simulink model "Palan_sim"  (R2019a)
settings: Solver=FixedStepDiscrete  StartTime=0.0  StopTime=inf  FixedStep=2e-4  RelTol=1e-3
PreLoadFcn:
  | waijung.modelPreload; % Required for working with Waijung Blockset. Do not remove.
undefined symbols (not defined in the file): CPHA_1Edge, CPOL_Low, disableTheCustomCode, DISTANCE_PER_TURN_X, Duplex, enableTheCustomCode, FirstBit_MSB, Full, HSEOSC, in1, initTheCustomCode, Link, LQFP64, modifySysTick, out1, outputCSHigh, outputCSLow, PPR_THETA, PPR_XY, PSC2V, ST, STM32F446RE, V2PSC, waitForPulse, xref
libraries: simulink x13, waijung_customcode x4, stm32f4_spi_lib x3, stm32f4_io_lib x2, stm32f4_device_config_lib x1
CloseFcn:
  | waijung.modelClose; % Required for working with Waijung Blockset. Do not remove.
settings Model: Creator=ELEPALAN  LastModifiedBy=ELE4202-200
settings OptimizationCC: DefaultParameterBehavior=Inlined  DefaultUnderspecifiedDataType=single  EnhancedBackFolding=on  PassReuseOutputArgsAs=Individual arguments  ZeroExternalMemoryAtStartup=off  ZeroInternalMemoryAtStartup=off  MaxStackSize=64  OptimizeBlockOrder=speed  DifferentSizesBufferReuse=on  OptimizationCustomize=off
settings DebuggingCC: ParameterTunabilityLossMsg=error  UnconnectedInputMsg=none  UnconnectedOutputMsg=none  UnconnectedLineMsg=none  SFMachineParentedDataDiag=error
settings HardwareCC: ProdBitPerPointer=32  ProdBitPerSizeT=32  ProdBitPerPtrDiffT=32  ProdLargestAtomicInteger=Long  ProdLargestAtomicFloat=Double  ProdWordSize=32  ProdLongLongMode=on  ProdHWDeviceType=ARM Compatible->ARM Cortex  TargetEndianess=LittleEndian
settings SFSimCC: MATLABDynamicMemAlloc=off
settings RTWCC: Description=STM32F4 Target  SystemTargetFile=stm32f4.tlc  GenerateMakefile=off  TemplateMakefile=ert_default_tmf  Toolchain=GNU Tools for ARM Embedded Processors
settings CodeAppCC: ForceParamTrailComments=on  IgnoreCustomStorageClasses=off  OperatorAnnotations=on  SimulinkDataObjDesc=on  SFDataObjDesc=on  InsertBlockDesc=on
settings STFCustomTargetCC: MultiwordLength=256  ModelReferenceCompliant=off  CombineOutputUpdateFcns=on  ERTCustomFileBanners=on  SupportContinuousTime=off  SupportNonInlinedSFcns=off  RemoveResetFunc=on  MATLABClassNameForMDSCustomization=Simulink.SoftwareTarget.ERTCustomization  GRTInterface=off  SystemTargetFile=stm32f4.tlc
settings ERTTargetCC: ModelReferenceCompliant=off  ParMdlRefBuildCompliant=off  CompOptLevelCompliant=off  ConcurrentExecutionCompliant=off  ModelStepFunctionPrototypeControlCompliant=off  CPPClassGenCompliant=off  UseToolchainInfoCompliant=off  InlinedParameterPlacement=NonHierarchical  ERTSrcFileBannerTemplate=stm32f4_code_template.cgt  ERTHdrFileBannerTemplate=stm32f4_code_template.cgt  ERTDataSrcFileTemplate=stm32f4_code_template.cgt  ERTDataHdrFileTemplate=stm32f4_code_template.cgt  ERTCustomFileTemplate=stm32f4_file_process.tlc

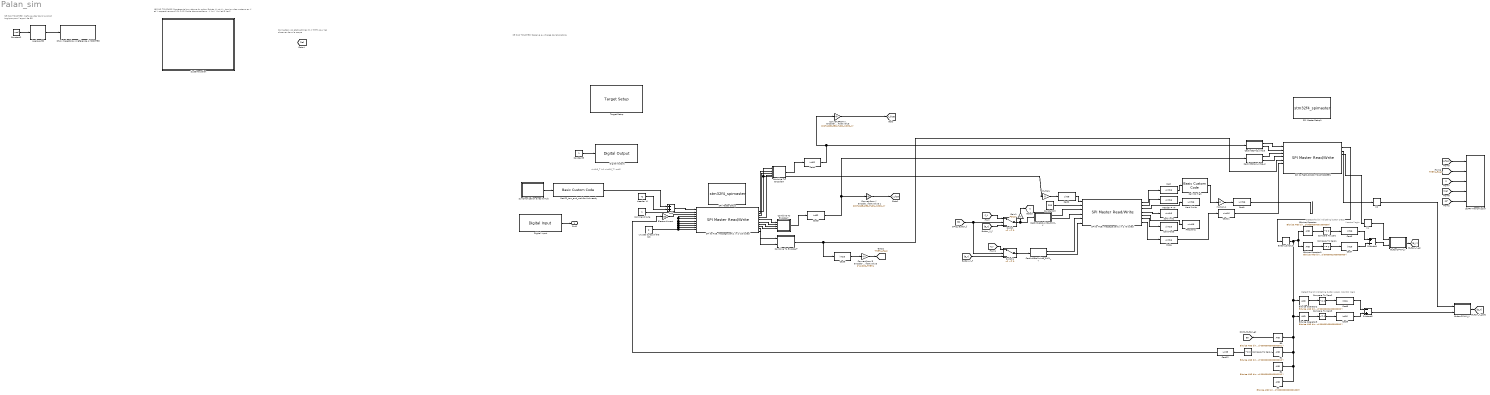
== system Palan_sim ==
  note: Detect the bit indicating button press.
  note: uint16_T in1,uint16_T* out1)
  note: NE PAS TOUCHER! Réservé au chargé de laboratoire
  note: Detect the bit indicating button press.
  note: Ycontrol logic
  note: Xcontrol logic
  note: NE PAS TOUCHER!
      | Xref à ajuster dans le script
      | Logique pour l'appui de B0
  note: Connectez vos états estimés [X,X',θ,θ'] pour les
      | observer dans le scope
  note: NE PAS TOUCHER!
      | Représente le système du palan
      | Entrée Vx et Vy: tension des moteurs en X et Y respectivement [-24,24]V
      | Sortie des encodeurs : X (m), Y(m) et θ (rad)
  Add : Sum  OutDataTypeStr=uint8  SaturateOnIntegerOverflow=on  InputSameDT=on
  B0 : simulink/Logic and Bit Operations/Bitwise Operator  logicop=AND  UseBitMask=on  BitMask=bin2dec('0000000000000001')  BitMaskRealWorld=Stored Integer
  B1 : simulink/Logic and Bit Operations/Bitwise Operator  logicop=AND  UseBitMask=on  BitMask=bin2dec('0000000000000010')  BitMaskRealWorld=Stored Integer
  B2 : simulink/Logic and Bit Operations/Bitwise Operator  logicop=AND  UseBitMask=on  BitMask=bin2dec('0000000000000100')  BitMaskRealWorld=Stored Integer
  B3 : simulink/Logic and Bit Operations/Bitwise Operator  logicop=AND  UseBitMask=on  BitMask=bin2dec('0000000000001000')  BitMaskRealWorld=Stored Integer
  Bitwise Operator : simulink/Logic and Bit Operations/Bitwise Operator  logicop=AND  UseBitMask=on  BitMask=bin2dec('0000000001000000')  BitMaskRealWorld=Stored Integer
  Bitwise Operator1 : simulink/Logic and Bit Operations/Bitwise Operator  logicop=AND  UseBitMask=on  BitMask=bin2dec('0000001000000000')  BitMaskRealWorld=Stored Integer
  Bitwise Operator2 : simulink/Logic and Bit Operations/Bitwise Operator  logicop=AND  UseBitMask=on  BitMask=bin2dec('0000000100000000')  BitMaskRealWorld=Stored Integer
  Bitwise Operator3 : simulink/Logic and Bit Operations/Bitwise Operator  logicop=AND  UseBitMask=on  BitMask=bin2dec('0000010000000000')  BitMaskRealWorld=Stored Integer
  Button2PWM_X : MATLAB Function  TreatAsAtomicUnit=on
  Button2PWM_Y : MATLAB Function  TreatAsAtomicUnit=on
  Button_Outputs : Memory
  CalibMode : DataTypeConversion  OutDataTypeStr=uint16
  Call CS High : waijung_customcode/Basic Custom Code  inputporttype=uint16  cinputportlabel=in1  cinputportlabelstr="[\"in1\"]"  inputportcount=1  inputporttypeid=[5]  outputporttype=uint16  coutputportlabel=ForceMeFirst  coutputportlabelstr="[\"ForceMeFirst\"]"  outputportcount=1  outputporttypeid=[5]  incpath={}  srcpath={fullfile(pwd,'customcode')}  incfiles={}  srcfiles={'customcode.c'}  initialfuncallstr=initTheCustomCode();  enablefuncallstr=enableTheCustomCode();  outputfuncallstr=outputCSHigh(in1,out1);  disablefuncallstr=disableTheCustomCode();  sampletime=2e-4  sampletimestr=-1  blockid=CallCSHigh  enablecustomportlabel=on  incfilestrarray=[]  inputportdiminfo="[1  1  1  5]"  outputportdiminfo="[1  1  1  5]"
      settings: SourceProductName=Waijung Blockset
  Cast : DataTypeConversion  OutDataTypeStr=uint16
  Cast1 : DataTypeConversion  OutDataTypeStr=uint16
  Cast11 : DataTypeConversion  OutDataTypeStr=uint16
  Cast12 : DataTypeConversion  OutDataTypeStr=uint8
  Cast2 : DataTypeConversion  OutDataTypeStr=uint8
  Cast{3,6..9} (5 alike) : DataTypeConversion  OutDataTypeStr=int16
  Cast4 : DataTypeConversion  OutDataTypeStr=int32
  Cast5 : DataTypeConversion  OutDataTypeStr=int32
  Castint16to2uint8_PWM_X : MATLAB Function  TreatAsAtomicUnit=on
  Castint16to2uint8_PWM_Y : MATLAB Function  TreatAsAtomicUnit=on
  Castint32To2uint16 : MATLAB Function  TreatAsAtomicUnit=on
  Castint32to2uint16_2 : MATLAB Function  TreatAsAtomicUnit=on
  Choix trajectoire vs référence À MODIFIER : Subsystem
  Combine To EncoderT : MATLAB Function  TreatAsAtomicUnit=on
  Combine To EncoderX : MATLAB Function  TreatAsAtomicUnit=on
  Combine To EncoderY : MATLAB Function  TreatAsAtomicUnit=on
  Commend byte : Constant  OutDataTypeStr=uint8  SampleTime=2e-4
  Compare To Zero{,1..4} (5 alike) : simulink/Logic and Bit Operations/Compare To Zero  relop=~=  OutDataTypeStr=boolean
  Constant13 : Constant  Value=255  OutDataTypeStr=uint8  SampleTime=2e-4
  Constant2 : Constant  Value=xref  SampleTime=-1
  Constant5 : Constant  OutDataTypeStr=boolean  SampleTime=2e-4
  "Convert FROM X encoder to X float value " : Gain  Gain=DISTANCE_PER_TURN_X/PPR_XY  OutDataTypeStr=single  SaturateOnIntegerOverflow=on  ParamDataTypeStr=Inherit: Same as input
  Convert from Y encoder to Y float value 1 : Gain  Gain=DISTANCE_PER_TURN_X/PPR_XY  OutDataTypeStr=single  SaturateOnIntegerOverflow=on  ParamDataTypeStr=Inherit: Same as input
  Convert from θ encoder to θ float value : Gain  Gain=2*pi/PPR_THETA  OutDataTypeStr=single  SaturateOnIntegerOverflow=on  ParamDataTypeStr=Inherit: Same as input
  Digital Input : stm32f4_io_lib/Digital Input  port=A  speed=100  porttype=None  porttypestr=NOPULL  use_pin0=on  use_pin1=off  use_pin2=off  use_pin3=off  use_pin4=off  use_pin5=off  use_pin6=off  use_pin7=off  use_pin8=off  use_pin9=off  use_pin10=off  use_pin11=off  use_pin12=off  use_pin13=off  use_pin14=off  use_pin15=off  pinstr=GPIO_Pin_0  usedpinarray="[1  0  0  0  0  0  0  0  0  0  0  0  0  0  0  0]"  bitbandingstr="#define DigitalInput_A0 Peripheral_BB(GPIOA->IDR, 0)  /* Output pin */"  sampletime=2e-4  sampletimestr=-1  blockid=DigitalInput  enablecustomportlabel=off  glabalinit=off  cinputportlabel=In1, In2  coutputportlabel=Out1, Out2
      settings: SourceProductName=Waijung Blockset
  Digital Output : stm32f4_io_lib/Digital Output  use_bitband=on  port=A  speed=100  porttype=Push Pull  porttypestr=PP  use_pin0=off  use_pin1=off  use_pin2=off  use_pin3=off  use_pin4=off  use_pin5=off  use_pin6=off  use_pin7=off  use_pin8=off  use_pin9=off  use_pin10=on  use_pin11=off  use_pin12=off  use_pin13=off  use_pin14=off  use_pin15=off  pinstr=GPIO_Pin_10  usedpinarray="[0  0  0  0  0  0  0  0  0  0  1  0  0  0  0  0]"  bitbandingstr="#define DigitalOutput_A10 Peripheral_BB(GPIOA->ODR, 10)  /* Output pin */"  sampletime=-1  sampletimestr=-1  blockid=DigitalOutput  enablecustomportlabel=off  globalinit=off  cinputportlabel=In1, In2  coutputportlabel=0
      settings: SourceProductName=Waijung Blockset
  Electro-Aimant : Gain  Gain=100  OutDataTypeStr=uint8  SaturateOnIntegerOverflow=on  ParamDataTypeStr=Inherit: Same as input
  Frequency : DataTypeConversion  OutDataTypeStr=uint16
  Gain1 : Gain  Gain=PSC2V  SaturateOnIntegerOverflow=on  OutDataTypeStr=Inherit: Same as input  ParamDataTypeStr=Inherit: Same as input
  Hard limits : DataTypeConversion  OutDataTypeStr=uint16
  Header 'H' : Constant  Value=72  OutDataTypeStr=uint8  SampleTime=2e-4
  Header = 'H' : DataTypeConversion  OutDataTypeStr=uint16
  K0 : Memory
  K1 : Memory
  Logique B0 : Subsystem
  Mode : DataTypeConversion  OutDataTypeStr=uint16
  Multiply : Gain  Gain=0  SaturateOnIntegerOverflow=on  OutDataTypeStr=Inherit: Same as input  ParamDataTypeStr=Inherit: Same as input
  Multiply1 : Gain  Gain=0  SaturateOnIntegerOverflow=on  OutDataTypeStr=Inherit: Same as input  ParamDataTypeStr=Inherit: Same as input
  SPI Master Setup : S-Function  FunctionName=stm32f4_spimaster  Parameters=mode,configuration,module,datacount,inputtypearray,outputtypearray,confstr,sampletime,sampletimestr,blockid  SFunctionDeploymentMode=off  EnableBusSupport=off  mask(stm32f4_spimaster){configuration=Setup, module=3, mode=Write, lastmodule=3, direction=Full-Duplex, dataformat=8bit/ FirstBit_MSB, prescaler=8, lastpclk=45000000, baudrate=5625000, cpolcpha=CPOL_Low/ CPHA_1Edge, datacount=0, nssmode=Software, nsspin=Not used, softnssport=B, softnsspin=10, sckpin=B3, misopin=B4, mosipin=B5, pintype=Push Pull, pulltype=None, nssdelay=0, inputtypearray=[0], outputtypearray=[0], confstr=["SPI_Direction_2Lines_FullDuplex","8b","MSB","Low","1Edge","8","Soft","0","x","x","1","B","10","1","B","3","1","B","4","1","B","5","0","1","0","0","0","0","0","0","0","PP","0","NOPULL"], sampletime=-1, sampletimestr=-1, blockid=SPIMasterSetup}
      mask prompts: module "SPI Module:"; lastmodule "Last module:"; dataformat "Data format:"; prescaler "Buad rate prescaler: Pclk/"; lastpclk "Last PCLK"; baudrate "Baud rate (Hz)"; cpolcpha "Clock polarity (CPOL)/ Clock phase (CPHA):"; datacount "Data Write count:"; nssmode "Slave/chip select (nSS, nCS) mode"; nsspin "Slave/chip select (nSS, nCS) pin"; softnssport "Slave/chip select port (nSS, nCS)"; softnsspin "Slave/chip select pin (nSS, nCS)"; sckpin "SCLK pin:"; misopin "MISO pin:"; mosipin "MOSI pin:"; pintype "Pin type (Push-Pull/Open-Drain)"; pulltype "Pull Type (Up/Down)"; nssdelay "Data delay time, uS:"; inputtypearray "Input type array"; outputtypearray "Output type array"; confstr "Configuration string"; sampletime "Sample time (sec)"; sampletimestr "Compiled sample time (sec) in string"
      mask help:
      | Direction:
      |  - Full-Duplex, use this mode when need to send and receive data at same clock.
      |  - Half-Duplex_Tx, this mode is to transmit data to slave only. Pin MISO (Rx) can be free for other function.
      |  - Half-Duplex_Rx, this mode is to receive data from slave only. Pin MOSIO (Tx) can be free for other function.
      | Data format:
      |   This configuration is depending on the specification of slave device.
      | Baud rate prescaler:
      |  - Use this prescaler to devide from the PCLK for SPI clock.
      |  - This Prescaler value is auto determine corresponding to baudrate setting and selected SPI module.
      | Baud rate (Hz):
      |  - Select baud rate for SPI clock. Please check the maximum clock support for target slave device.
      | Clock polarity and Clock phase:
      |  - This configuration parameter is depending on slave device.
      |  - See waijung help for more description.
      | Slave/chip select mode:
      |  - Hardware, use hardware SPI module for slave select (or chip select) pin.
      |  - Software, this mode allow any available pin for slave select (or chip select) function.
      |  - Custom, SPI block did not control slave select pin. User may use Digital Output block to control by costom.
      mask init:
      | stm32f4_spimaster_callback('init');
      mask Help: web(fullfile(waijungdocroot,'stm32f4_spimaster_setup.htm'), '-browser')
      mask TypeOptions configuration: Setup | Transaction
      mask Callback configuration: stm32f4_spimaster_callback('configuration');
      mask TypeOptions module: 1 | 2 | 3
      mask Callback module: stm32f4_spimaster_callback('module');
      mask TypeOptions mode: Read/ Write | Read | Write
      mask Callback mode: stm32f4_spimaster_callback('mode');
      mask TypeOptions direction: Full-Duplex | Half-Duplex_Tx | Half-Duplex_Rx
      mask Callback direction: stm32f4_spimaster_callback('direction');
      mask TypeOptions dataformat: 8bit/ FirstBit_MSB | 8bit/ FirstBit_LSB | 16bit/ FirstBit_MSB | 16bit/ FirstBit_LSB
      mask TypeOptions prescaler: 2 | 4 | 8 | 16 | 32 | 64 | 128 | 256
      mask TypeOptions baudrate: Not set | 22500000 | 11250000 | 5625000 | 2812500 | 1406250 | 703125 | 351563 | 175781
      mask Callback baudrate: stm32f4_spimaster_callback('baudrate');
      mask TypeOptions cpolcpha: CPOL_Low/ CPHA_1Edge | CPOL_Low/ CPHA_2Edge | CPOL_High/ CPHA_1Edge | CPOL_High/ CPHA_2Edge
      mask Callback datacount: stm32f4_spimaster_callback('datacount');
      mask TypeOptions nssmode: Hardware | Software | Custom
      mask Callback nssmode: stm32f4_spimaster_callback('nssmode');
      mask TypeOptions nsspin: Not used | A4
      mask TypeOptions softnssport: A | B | C | D | E | F | G | H | I
      mask TypeOptions softnsspin: 0 | 1 | 2 | 3 | 4 | 5 | 6 | 7 | 8 | 9 | 10 | 11 | 12 | 13 | 14 | 15
      mask TypeOptions sckpin: Not used | B3 | C10
      mask TypeOptions misopin: Not used | B4 | C11
      mask TypeOptions mosipin: Not used | B5 | C12
      mask TypeOptions pintype: Push Pull | Open Drain
      mask TypeOptions pulltype: None | Pull Up | Pull Down
      mask Callback confstr: stm32f4_spimaster_callback('confstr');
      mask Callback sampletime: stm32f4_spimaster_callback('sampletime');
      mask Callback sampletimestr: stm32f4_spimaster_callback('sampletimestr');
      mask Callback blockid: stm32f4_spimaster_callback('blockid');
      mask Display: text(0.5, 0.5, 'Module: SPI3 (Master)\nFull-Duplex\nBaudrate: 5625000','ver','middle','hor','center');
  SPI Master Setup1 : S-Function  FunctionName=stm32f4_spimaster  Parameters=mode,configuration,module,datacount,inputtypearray,outputtypearray,confstr,sampletime,sampletimestr,blockid  SFunctionDeploymentMode=off  EnableBusSupport=off  mask(stm32f4_spimaster){configuration=Setup, module=1, mode=Write, lastmodule=1, direction=Full-Duplex, dataformat=16bit/ FirstBit_MSB, prescaler=8, lastpclk=90000000, baudrate=11250000, cpolcpha=CPOL_Low/ CPHA_1Edge, datacount=0, nssmode=Software, nsspin=Not used, softnssport=B, softnsspin=6, sckpin=A5, misopin=A6, mosipin=A7, pintype=Push Pull, pulltype=Pull Up, nssdelay=0, inputtypearray=[0], outputtypearray=[0], confstr=["SPI_Direction_2Lines_FullDuplex","16b","MSB","Low","1Edge","8","Soft","0","x","x","1","B","6","1","A","5","1","A","6","1","A","7","1","1","0","0","0","0","0","0","0","PP","0","UP"], sampletime=-1, sampletimestr=-1, blockid=SPIMasterSetup1}
      mask prompts: module "SPI Module:"; lastmodule "Last module:"; dataformat "Data format:"; prescaler "Buad rate prescaler: Pclk/"; lastpclk "Last PCLK"; baudrate "Baud rate (Hz)"; cpolcpha "Clock polarity (CPOL)/ Clock phase (CPHA):"; datacount "Data Write count:"; nssmode "Slave/chip select (nSS, nCS) mode"; nsspin "Slave/chip select (nSS, nCS) pin"; softnssport "Slave/chip select port (nSS, nCS)"; softnsspin "Slave/chip select pin (nSS, nCS)"; sckpin "SCLK pin:"; misopin "MISO pin:"; mosipin "MOSI pin:"; pintype "Pin type (Push-Pull/Open-Drain)"; pulltype "Pull Type (Up/Down)"; nssdelay "Data delay time, uS:"; inputtypearray "Input type array"; outputtypearray "Output type array"; confstr "Configuration string"; sampletime "Sample time (sec)"; sampletimestr "Compiled sample time (sec) in string"
      mask help:
      | Direction:
      |  - Full-Duplex, use this mode when need to send and receive data at same clock.
      |  - Half-Duplex_Tx, this mode is to transmit data to slave only. Pin MISO (Rx) can be free for other function.
      |  - Half-Duplex_Rx, this mode is to receive data from slave only. Pin MOSIO (Tx) can be free for other function.
      | Data format:
      |   This configuration is depending on the specification of slave device.
      | Baud rate prescaler:
      |  - Use this prescaler to devide from the PCLK for SPI clock.
      |  - This Prescaler value is auto determine corresponding to baudrate setting and selected SPI module.
      | Baud rate (Hz):
      |  - Select baud rate for SPI clock. Please check the maximum clock support for target slave device.
      | Clock polarity and Clock phase:
      |  - This configuration parameter is depending on slave device.
      |  - See waijung help for more description.
      | Slave/chip select mode:
      |  - Hardware, use hardware SPI module for slave select (or chip select) pin.
      |  - Software, this mode allow any available pin for slave select (or chip select) function.
      |  - Custom, SPI block did not control slave select pin. User may use Digital Output block to control by costom.
      mask init:
      | stm32f4_spimaster_callback('init');
      mask Help: web(fullfile(waijungdocroot,'stm32f4_spimaster_setup.htm'), '-browser')
      mask TypeOptions configuration: Setup | Transaction
      mask Callback configuration: stm32f4_spimaster_callback('configuration');
      mask TypeOptions module: 1 | 2 | 3
      mask Callback module: stm32f4_spimaster_callback('module');
      mask TypeOptions mode: Read/ Write | Read | Write
      mask Callback mode: stm32f4_spimaster_callback('mode');
      mask TypeOptions direction: Full-Duplex | Half-Duplex_Tx | Half-Duplex_Rx
      mask Callback direction: stm32f4_spimaster_callback('direction');
      mask TypeOptions dataformat: 8bit/ FirstBit_MSB | 8bit/ FirstBit_LSB | 16bit/ FirstBit_MSB | 16bit/ FirstBit_LSB
      mask TypeOptions prescaler: 2 | 4 | 8 | 16 | 32 | 64 | 128 | 256
      mask TypeOptions baudrate: Not set | 45000000 | 22500000 | 11250000 | 5625000 | 2812500 | 1406250 | 703125 | 351563 | 5250000
      mask Callback baudrate: stm32f4_spimaster_callback('baudrate');
      mask TypeOptions cpolcpha: CPOL_Low/ CPHA_1Edge | CPOL_Low/ CPHA_2Edge | CPOL_High/ CPHA_1Edge | CPOL_High/ CPHA_2Edge
      mask Callback datacount: stm32f4_spimaster_callback('datacount');
      mask TypeOptions nssmode: Hardware | Software | Custom
      mask Callback nssmode: stm32f4_spimaster_callback('nssmode');
      mask TypeOptions nsspin: Not used | A4 | A15
      mask TypeOptions softnssport: A | B | C | D | E | F | G | H | I
      mask TypeOptions softnsspin: 0 | 1 | 2 | 3 | 4 | 5 | 6 | 7 | 8 | 9 | 10 | 11 | 12 | 13 | 14 | 15
      mask TypeOptions sckpin: Not used | A5 | B3
      mask TypeOptions misopin: Not used | A6 | B4
      mask TypeOptions mosipin: Not used | A7 | B5
      mask TypeOptions pintype: Push Pull | Open Drain
      mask TypeOptions pulltype: None | Pull Up | Pull Down
      mask Callback confstr: stm32f4_spimaster_callback('confstr');
      mask Callback sampletime: stm32f4_spimaster_callback('sampletime');
      mask Callback sampletimestr: stm32f4_spimaster_callback('sampletimestr');
      mask Callback blockid: stm32f4_spimaster_callback('blockid');
      mask Display: text(0.5, 0.5, 'Module: SPI1 (Master)\nFull-Duplex\nBaudrate: 11250000','ver','middle','hor','center');
  SPI to F469I-DISCO TOUCHSCREEN : stm32f4_spi_lib/SPI Master Read//Write  configuration=Transaction  module=1  mode=Read/ Write  lastmodule=1  direction=Full-Duplex  dataformat=16bit/ FirstBit_MSB  prescaler=4  cpolcpha=CPOL_Low/ CPHA_1Edge  datacount=8  nssmode=Custom  nsspin=Not used  softnssport=E  softnsspin=0  sckpin=A5  misopin=A6  mosipin=A7  inputtypearray=[8 5 5 5 5 5 5 5 5]  outputtypearray=[9 7 5 5 5 5 5 5 5 5]  confstr="[\"SPI_Direction_2Lines_FullDuplex\",\"16b\",\"MSB\",\"Low\",\"1Edge\",\"4\",\"Soft\",\"0\",\"x\",\"x\",\"0\",\"x\",\"x\",\"1\",\"A\",\"5\",\"1\",\"A\",\"6\",\"1\",\"A\",\"7\",\"1\",\"0\",\"0\",\"0\",\"0\",\"0\",\"0\",\"0\",\"0\",\"PP\",\"0\",\"UP\"]"  sampletime=2e-4  sampletimestr=-1  blockid=SPItoF469IDISCOTOUCHSCREEN
      settings: SourceProductName=Waijung Blockset
  "SPI to HUB, message part 1 in 2 (10 bytes)" : stm32f4_spi_lib/SPI Master Read//Write  configuration=Transaction  module=3  mode=Read/ Write  lastmodule=1  direction=Full-Duplex  dataformat=8bit/ FirstBit_MSB  prescaler=4  cpolcpha=CPOL_Low/ CPHA_1Edge  datacount=10  nssmode=Custom  nsspin=Not used  softnssport=E  softnsspin=0  sckpin=A5  misopin=A6  mosipin=A7  inputtypearray=[10 3 3 3 3 3 3 3 3 3 3]  outputtypearray=[11 7 3 3 3 3 3 3 3 3 3 3]  confstr="[\"SPI_Direction_2Lines_FullDuplex\",\"8b\",\"MSB\",\"Low\",\"1Edge\",\"4\",\"Soft\",\"0\",\"x\",\"x\",\"0\",\"x\",\"x\",\"1\",\"A\",\"5\",\"1\",\"A\",\"6\",\"1\",\"A\",\"7\",\"1\",\"0\",\"0\",\"0\",\"0\",\"0\",\"0\",\"0\",\"0\",\"PP\",\"0\",\"UP\"]"  sampletime=2e-4  sampletimestr=-1  blockid=SPItoHUBmessagepart1in210bytes
      settings: SourceProductName=Waijung Blockset
  "SPI to HUB, message part 2 in 2 (6 bytes)" : stm32f4_spi_lib/SPI Master Read//Write  configuration=Transaction  module=3  mode=Read/ Write  lastmodule=1  direction=Full-Duplex  dataformat=8bit/ FirstBit_MSB  prescaler=4  cpolcpha=CPOL_Low/ CPHA_1Edge  datacount=6  nssmode=Custom  nsspin=Not used  softnssport=E  softnsspin=0  sckpin=A5  misopin=A6  mosipin=A7  inputtypearray=[6 3 3 3 3 3 3]  outputtypearray=[7 7 3 3 3 3 3 3]  confstr="[\"SPI_Direction_2Lines_FullDuplex\",\"8b\",\"MSB\",\"Low\",\"1Edge\",\"4\",\"Soft\",\"0\",\"x\",\"x\",\"0\",\"x\",\"x\",\"1\",\"A\",\"5\",\"1\",\"A\",\"6\",\"1\",\"A\",\"7\",\"1\",\"0\",\"0\",\"0\",\"0\",\"0\",\"0\",\"0\",\"0\",\"PP\",\"0\",\"UP\"]"  sampletime=2e-4  sampletimestr=-1  blockid=SPItoHUBmessagepart2in26bytes
      settings: SourceProductName=Waijung Blockset
  Set CS_Low_and_wait for Hub ready : waijung_customcode/Basic Custom Code  inputporttype=uint16  cinputportlabel=in1  cinputportlabelstr="[\"in1\"]"  inputportcount=1  inputporttypeid=[5]  outputporttype=uint16  coutputportlabel=ForceMeFirst  coutputportlabelstr="[\"ForceMeFirst\"]"  outputportcount=1  outputporttypeid=[5]  incpath={}  srcpath={fullfile(pwd,'customcode')}  incfiles={}  srcfiles={'customcode.c'}  initialfuncallstr=initTheCustomCode();  enablefuncallstr=enableTheCustomCode();  outputfuncallstr=outputCSLow(in1, out1);  disablefuncallstr=disableTheCustomCode();  sampletime=2e-4  sampletimestr=-1  blockid=SetCS_Low_and_waitforHubready  enablecustomportlabel=on  incfilestrarray=[]  inputportdiminfo="[1  1  1  5]"  outputportdiminfo="[1  1  1  5]"
      settings: SourceProductName=Waijung Blockset
  Soft limits : DataTypeConversion  OutDataTypeStr=uint16
  Subtract1 : Sum  Inputs=+-  SaturateOnIntegerOverflow=on  InputSameDT=on  OutDataTypeStr=Inherit: Same as first input
  Subtract2 : Sum  Inputs=-+  SaturateOnIntegerOverflow=on  InputSameDT=on  OutDataTypeStr=Inherit: Same as first input
  Switch : Switch  Criteria=u2 ~= 0  OutDataTypeStr=int32
  Switch1 : Switch  Criteria=u2 ~= 0  OutDataTypeStr=int32
  Synchronisation avec le Hub : Subsystem
  Système palan : Subsystem
  Target Setup : stm32f4_device_config_lib/Target Setup  Priority=100  compiler=GNU ARM  previous_compiler=GNU ARM  mcu=STM32F446RE (LQFP64)  mcustr=STM32F446RE  clockconfig=HSEOSC-8MHz  system_stm32f4xx_c_path=C:\Palans\workspace\ELE3200_Banc_Moteur\waijung_18.11a\targets\stm32f4_target\stm32f4\utils\system_stm32f4xx_default\STM32F446xx\hseosc8mhz  showmemoryconfiguration=off  stacksize=0x2000  heapsize=0x2000  enableautocompiledownload=on  fullchiperase=off  programmerinterface=ST-Link  editctrlstr=on  compilercontrolstr=$(patsubst %, -I%, .) -mcpu=cortex-m4 -mthumb -mthumb-interwork -mfloat-abi=hard -mfpu=fpv4-sp-d16 -ffast-math -Wall -Wextra -Ofast  assemblercontrolstr=$(patsubst %, -I%, .) -mcpu=cortex-m4 -mthumb -mthumb-interwork -mfloat-abi=hard -mfpu=fpv4-sp-d16 -ffast-math -Wall -Wextra -Ofast -Wa,-amhls=$(<:.s=.lst) -D__STACK_SIZE=$(STACK_SIZE) -D__HEAP_SIZE=$(HEAP_SIZE)  linkercontrolstr=-T$(LD_SCRIPT) -g -Wl,-Map=$(MAP),--cref,--no-warn-mismatch -mcpu=cortex-m4 -mthumb -mthumb-interwork -mfloat-abi=hard -mfpu=fpv4-sp-d16 -specs=nosys.specs  runafterdownload=on  execprofile=None  profileruart=2  profilerbaud=500000  profilertxpin=A2  profilerinitstr=2e-4,180000000,36000,500000,0  manualsetsampletime=on  sampletime=2e-4  blockid=TargetSetup  systickreloadvalue=36000  hseval=8000000  lastprofileruart=2  hclk=180000000  flashorigin=0x8000000  flashlength=512k  ramorigin=0x20000000  ramlength=128k  useextram=off
      settings: SourceProductName=Waijung Blockset
  USART Transmission : Subsystem  Description="Blok envoyant les données par UART pour qu'elles soient lues et enregistrées par l'ordianteur via le modèle simulink \"Host\""
  unused bytes of the SPI : Constant  Value=0  OutDataTypeStr=uint8  SampleTime=2e-4
  Out1 : Outport
  tag scope: B0=global, THETA_float=global, U=global, X_float=global, Y_float=global
  wires:
  Digital Input/1 -> Out1/1
  Subtract1/1 -> Button2PWM_Y/2(u)
  SPI to F469I-DISCO TOUCHSCREEN/3 -> K0/1
  "SPI to HUB, message part 1 in 2 (10 bytes)"/2 -> Combine To EncoderX/1(u1), Multiply/1
  [B_X] -> Switch/3
  Combine To EncoderX/1(x) -> Cast4/1
  "SPI to HUB, message part 2 in 2 (6 bytes)"/1 -> Cast/1
  Convert from θ encoder to θ float value/1 -> [THETA_float]
  Compare To Zero3/1 -> Cast9/1
  Button2PWM_Y/1(y) -> [B_Y]
  B0/1 -> [B0]
  "SPI to HUB, message part 1 in 2 (10 bytes)"/4 -> Combine To EncoderX/3(u3)
  Castint16to2uint8_PWM_X/2(x2) -> "SPI to HUB, message part 2 in 2 (6 bytes)"/4
  Castint32to2uint16_2/2(y) -> SPI to F469I-DISCO TOUCHSCREEN/4
  Cast1/1 -> ?
  "SPI to HUB, message part 1 in 2 (10 bytes)"/3 -> Combine To EncoderX/2(u2)
  [F_Y] -> Switch1/1
  "Convert FROM X encoder to X float value "/1 -> [X_float]
  [B_Y] -> Switch1/3
  Cast7/1 -> Subtract1/2
  Multiply1/1 -> Cast1/1
  B1/1 -> Compare To Zero4/1
  Castint16to2uint8_PWM_Y/1(x1) -> "SPI to HUB, message part 2 in 2 (6 bytes)"/5
  Cast12/1 -> Electro-Aimant/1
  Bitwise Operator3/1 -> Compare To Zero3/1
  Header 'H'/1 -> Add/2
  Compare To Zero/1 -> Cast3/1
  Combine To EncoderT/1(x) -> SPI to F469I-DISCO TOUCHSCREEN/5, Cast6/1
  Multiply/1 -> Cast2/1
  Constant5/1 -> Digital Output/1
  "SPI to HUB, message part 1 in 2 (10 bytes)"/8 -> Combine To EncoderY/3(u3)
  Combine To EncoderY/1(x) -> Cast5/1
  "SPI to HUB, message part 1 in 2 (10 bytes)"/9 -> Combine To EncoderY/4(u4)
  "SPI to HUB, message part 2 in 2 (6 bytes)"/3 -> Hard limits/1
  "SPI to HUB, message part 1 in 2 (10 bytes)"/11 -> Combine To EncoderT/2(u2)
  Cast3/1 -> Subtract1/1
  "SPI to HUB, message part 2 in 2 (6 bytes)"/6 -> CalibMode/1
  Set CS_Low_and_wait for Hub ready/1 -> Add/1  "0"
  "SPI to HUB, message part 2 in 2 (6 bytes)"/5 -> Frequency/1
  SPI to F469I-DISCO TOUCHSCREEN/2 -> Button_Outputs/1
  Button_Outputs/1 -> Bitwise Operator/1, Bitwise Operator1/1, B2/1, B3/1, B1/1, B0/1, Bitwise Operator3/1, Bitwise Operator2/1
  "SPI to HUB, message part 2 in 2 (6 bytes)"/2 -> Header = 'H'/1
  Cast2/1 -> "SPI to HUB, message part 2 in 2 (6 bytes)"/1
  K0/1 -> Button2PWM_X/1(K)
  "SPI to HUB, message part 1 in 2 (10 bytes)"/5 -> Combine To EncoderX/4(u4)
  Button2PWM_X/1(y) -> [B_X]
  Bitwise Operator1/1 -> Compare To Zero1/1
  Cast5/1 -> Castint32to2uint16_2/1(u), Convert from Y encoder to Y float value 1/1
  [B0] -> Switch1/2, Switch/2
  Subtract2/1 -> Button2PWM_X/2(u)
  Cast9/1 -> Subtract2/2
  "SPI to HUB, message part 1 in 2 (10 bytes)"/7 -> Combine To EncoderY/2(u2)
  Bitwise Operator/1 -> Compare To Zero/1
  Castint32To2uint16/1(x) -> SPI to F469I-DISCO TOUCHSCREEN/1
  Electro-Aimant/1 -> "SPI to HUB, message part 1 in 2 (10 bytes)"/3
  "SPI to HUB, message part 2 in 2 (6 bytes)"/4 -> Soft limits/1
  Call CS High/1 -> Multiply1/1
  Castint32to2uint16_2/1(x) -> SPI to F469I-DISCO TOUCHSCREEN/3
  Compare To Zero2/1 -> Cast8/1
  Cast/1 -> Call CS High/1
  "SPI to HUB, message part 2 in 2 (6 bytes)"/7 -> Mode/1
  [F_X] -> Switch/1
  Cast11/1 -> SPI to F469I-DISCO TOUCHSCREEN/6
  "SPI to HUB, message part 1 in 2 (10 bytes)"/10 -> Combine To EncoderT/1(u1)
  unused bytes of the SPI/1 -> "SPI to HUB, message part 1 in 2 (10 bytes)"/9, "SPI to HUB, message part 1 in 2 (10 bytes)"/7, "SPI to HUB, message part 1 in 2 (10 bytes)"/6, "SPI to HUB, message part 1 in 2 (10 bytes)"/5, "SPI to HUB, message part 1 in 2 (10 bytes)"/4, "SPI to HUB, message part 1 in 2 (10 bytes)"/8, "SPI to HUB, message part 1 in 2 (10 bytes)"/10
  Castint32To2uint16/2(y) -> SPI to F469I-DISCO TOUCHSCREEN/2
  Switch1/1 -> Castint16to2uint8_PWM_Y/1(u)
  Convert from Y encoder to Y float value 1/1 -> [Y_float]
  "SPI to HUB, message part 1 in 2 (10 bytes)"/6 -> Combine To EncoderY/1(u1)
  Cast8/1 -> Subtract2/1
  Constant13/1 -> "SPI to HUB, message part 2 in 2 (6 bytes)"/2
  Castint16to2uint8_PWM_Y/2(x2) -> "SPI to HUB, message part 2 in 2 (6 bytes)"/6
  Bitwise Operator2/1 -> Compare To Zero2/1
  Compare To Zero4/1 -> Cast12/1
  Castint16to2uint8_PWM_X/1(x1) -> "SPI to HUB, message part 2 in 2 (6 bytes)"/3
  Commend byte/1 -> "SPI to HUB, message part 1 in 2 (10 bytes)"/2
  Switch/1 -> Gain1/1, Castint16to2uint8_PWM_X/1(u)
  Compare To Zero1/1 -> Cast7/1
  Synchronisation avec le Hub/1(Out2) -> Set CS_Low_and_wait for Hub ready/1
  Add/1 -> "SPI to HUB, message part 1 in 2 (10 bytes)"/1
  Cast4/1 -> "Convert FROM X encoder to X float value "/1, Castint32To2uint16/1(u)
  K1/1 -> Button2PWM_Y/1(K)
  Mode/1 -> Cast11/1
  SPI to F469I-DISCO TOUCHSCREEN/4 -> K1/1
  Gain1/1 -> [U]
  Cast6/1 -> Convert from θ encoder to θ float value/1
  [U] -> USART Transmission/3(U)
  [X_float] -> USART Transmission/1(X)
  [THETA_float] -> USART Transmission/2(Theta)
  [Xe] -> USART Transmission/4(Xe)
  [ref] -> USART Transmission/5(Ref)
  Logique B0/1(Xref1) -> Choix trajectoire vs référence À MODIFIER/1(Xref)
  Constant2/1 -> Logique B0/1(Xref)

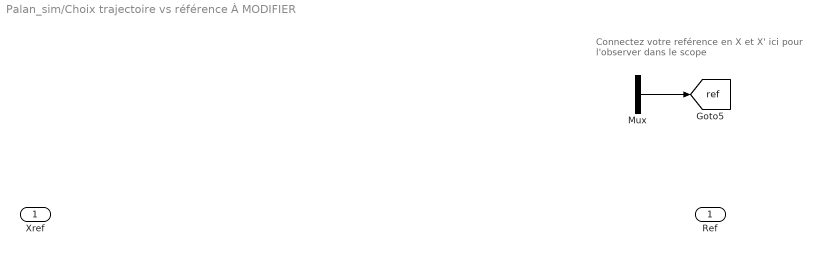
== system Palan_sim/Choix trajectoire vs référence À MODIFIER ==
  note: Connectez votre reférence en X et X' ici pour
      | l'observer dans le scope
  Xref : Inport
  Mux : Mux  Inputs=2
  Ref : Outport
  tag scope: ref=global
  wires:
  Mux/1 -> [ref]

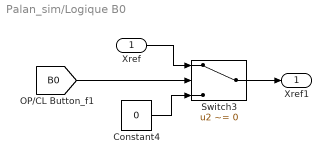
== system Palan_sim/Logique B0 ==
  Xref : Inport
  Constant4 : Constant  Value=0  SampleTime=-1
  Switch3 : Switch  Criteria=u2 ~= 0
  Xref1 : Outport
  wires:
  [B0] -> Switch3/2
  Constant4/1 -> Switch3/3
  Xref/1 -> Switch3/1
  Switch3/1 -> Xref1/1

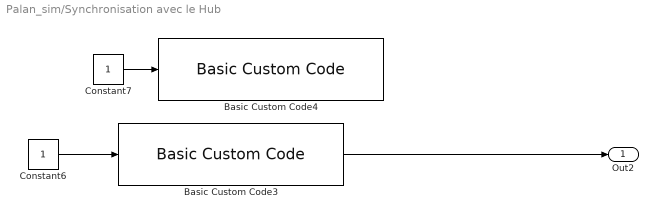
== system Palan_sim/Synchronisation avec le Hub ==
  Basic Custom Code3 : waijung_customcode/Basic Custom Code  inputporttype=uint16  cinputportlabel=in1  cinputportlabelstr="[\"in1\"]"  inputportcount=1  inputporttypeid=[5]  outputporttype=uint16  coutputportlabel=ForceMeFirst  coutputportlabelstr="[\"ForceMeFirst\"]"  outputportcount=1  outputporttypeid=[5]  incpath={}  srcpath={fullfile(pwd,'customcode')}  incfiles={}  srcfiles={'customcode.c'}  initialfuncallstr=initTheCustomCode();  enablefuncallstr=enableTheCustomCode();  outputfuncallstr=waitForPulse(in1, out1);  disablefuncallstr=disableTheCustomCode();  sampletime=2e-4  sampletimestr=-1  blockid=SynchronisationavecleHubBasicCustomCode3  enablecustomportlabel=on  incfilestrarray=[]  inputportdiminfo="[1  1  1  5]"  outputportdiminfo="[1  1  1  5]"
      settings: SourceProductName=Waijung Blockset
  Basic Custom Code4 : waijung_customcode/Basic Custom Code  inputporttype=uint16  cinputportlabel=in1  cinputportlabelstr="[\"in1\"]"  inputportcount=1  inputporttypeid=[5]  outputporttype=uint16  coutputportlabel=ModifySysTick  coutputportlabelstr="[\"ModifySysTick\"]"  outputportcount=1  outputporttypeid=[5]  incpath={}  srcpath={fullfile(pwd,'customcode')}  incfiles={}  srcfiles={'customcode.c'}  initialfuncallstr=initTheCustomCode();  enablefuncallstr=enableTheCustomCode();  outputfuncallstr=modifySysTick(in1, out1);  disablefuncallstr=disableTheCustomCode();  sampletime=-1  sampletimestr=-1  blockid=SynchronisationavecleHubBasicCustomCode4  enablecustomportlabel=on  incfilestrarray=[]  inputportdiminfo="[1  1  1  5]"  outputportdiminfo="[1  1  1  5]"
      settings: SourceProductName=Waijung Blockset
  Constant6 : Constant  OutDataTypeStr=uint16  SampleTime=2e-4
  Constant7 : Constant  OutDataTypeStr=uint16  SampleTime=2e-4
  Out2 : Outport
  wires:
  Constant7/1 -> Basic Custom Code4/1
  Constant6/1 -> Basic Custom Code3/1
  Basic Custom Code3/1 -> Out2/1

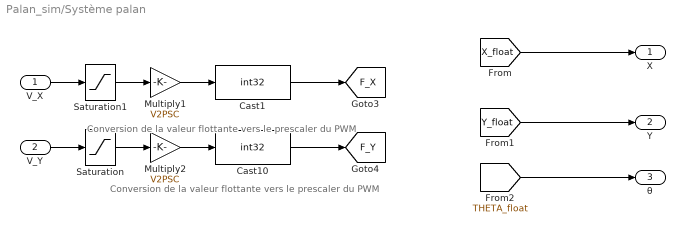
== system Palan_sim/Système palan ==
  note: Conversion de la valeur flottante vers le prescaler du PWM
  note: Conversion de la valeur flottante vers le prescaler du PWM
  V_X : Inport
  V_Y : Inport  Port=2
  Cast1 : DataTypeConversion  OutDataTypeStr=int32
  Cast10 : DataTypeConversion  OutDataTypeStr=int32
  Multiply1 : Gain  Gain=V2PSC  ParamDataTypeStr=single  OutDataTypeStr=single  SaturateOnIntegerOverflow=on
  Multiply2 : Gain  Gain=V2PSC  ParamDataTypeStr=single  OutDataTypeStr=single  SaturateOnIntegerOverflow=on
  Saturation : Saturate  UpperLimit=24  LowerLimit=-24
  Saturation1 : Saturate  UpperLimit=24  LowerLimit=-24
  X : Outport
  Y : Outport  Port=2
  θ : Outport  Port=3
  tag scope: F_X=global, F_Y=global
  wires:
  [X_float] -> X/1
  [Y_float] -> Y/1
  Multiply2/1 -> Cast10/1
  Cast10/1 -> [F_Y]
  Saturation/1 -> Multiply2/1
  V_Y/1 -> Saturation/1
  Multiply1/1 -> Cast1/1
  Cast1/1 -> [F_X]
  Saturation1/1 -> Multiply1/1
  V_X/1 -> Saturation1/1
  [THETA_float] -> θ/1

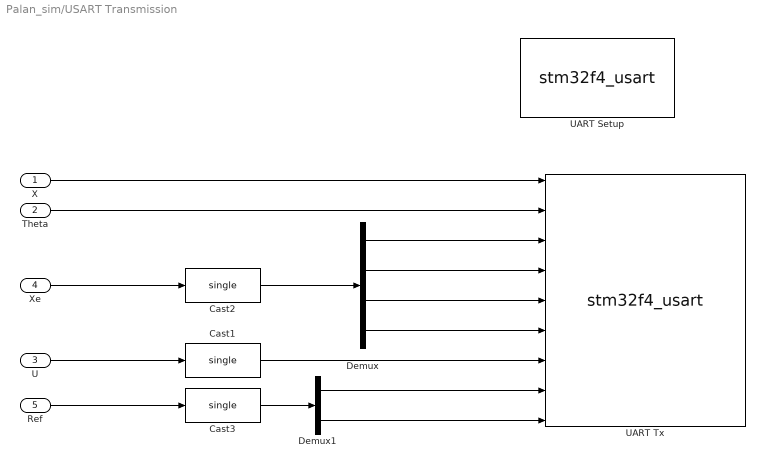
== system Palan_sim/USART Transmission ==
  X : Inport
  Theta : Inport  Port=2
  U : Inport  Port=3
  Xe : Inport  Port=4
  Ref : Inport  Port=5
  Cast1 : DataTypeConversion  OutDataTypeStr=single
  Cast2 : DataTypeConversion  OutDataTypeStr=single
  Cast3 : DataTypeConversion  OutDataTypeStr=single
  Demux : Demux
  Demux1 : Demux  Outputs=2
  UART Setup : S-Function  Priority=1  FunctionName=stm32f4_usart  Parameters=configuration,uartmodule,transfer,baudrate,inputtype,outputtype,confstr,binheaderarray,binterminatorarray,asciiheader,asciiterminator,bindatalength,packetmode,varname,sampletime,sampletimestr,blockid  SFunctionDeploymentMode=off  EnableBusSupport=off  mask(stm32f4_usart){configuration=Setup, uartmodule=2, baudrate=5500000, databits=8, parity=No, stopbit=1, remaptxpin=A2, remaprxpin=A3, flowcontrol=None, remapctspin=Not used, remaprtspin=Not used, advanceoptions=on, rxbuffersize=1024, txbuffersize=1024, transfer=Blocking, packetmode=Ascii, binheader='7E 7E', binterminator='03 03', porttype_double=1, porttype_single=0, porttype_int8=1, porttype_uint8=0, porttype_int16=0, porttype_uint16=0, porttype_int32=0, porttype_uint32=0, asciiformat='%d,%f', rx_asciiterminator=CRLF (0x0D 0x0A - "\r\n"), tx_asciiterminator=CR (0x0D - "\r"), storagename=<empty>, varname=, inputtype=[0], outputtype=[0], binheaderarray=[0], binterminatorarray=[0], bindatalength=0, asciiheader='', asciiterminator=[0], sampletime=-1, sampletimestr=-1, blockid=USARTTransmissionUARTSetup, confstr=[ "dummy", "1", "A", "2", "1", "A", "3", "0", "*", "*", "0", "*", "*", "1", "4", "6", "1", "4", "5", "1024", "1024", "1", "2", "5500000", "8", "No", "1", "None", "USART2"], lastmodule=2}
      mask prompts: uartmodule "UART Module"; baudrate "Baud rate (bps)"; databits "Data bits"; stopbit "Stop bit"; remaptxpin "Tx Pin"; remaprxpin "Rx Pin"; flowcontrol "Hardware flow control"; remapctspin "HW Flow control, CTS Pin"; remaprtspin "HW Flow control, RTS Pin"; advanceoptions "Advance options"; rxbuffersize "Rx buffer size (bytes)"; txbuffersize "Tx buffer size (bytes)"; packetmode "Packet mode"; binheader "Binary header (example: '7E 7E')"; binterminator "Binary terminator (example: '03 03')"; porttype_double "Number of data port, type DOUBLE"; porttype_single "Number of data port, type SINGLE"; porttype_int8 "Number of data port, type INT8"; porttype_uint8 "Number of data port, type UINT8"; porttype_int16 "Number of data port, type INT16"; porttype_uint16 "Number of data port, type UINT16"; porttype_int32 "Number of data port, type INT32"; porttype_uint32 "Number of data port, type UINT32"; asciiformat "Ascii format"; rx_asciiterminator "End of packet"; tx_asciiterminator "End of packet"; storagename "Buffer"; varname "Var name"; inputtype "Input data type"; outputtype "Output data type"; binheaderarray "Binary header"; binterminatorarray "Binary terminator"; bindatalength "Binary data length"; asciiheader "Ascii header (printf format)"; asciiterminator "Ascii terminator"; sampletime "Sample time (sec)"; sampletimestr "Compiled sample time (sec) in string"; confstr "Configuration string"; lastmodule "Last module selected"
      mask help:
      | Default STM32F4DISCOVERY + aMG F4 Connect 2 + aMG USB Converter N2 settings use
      |
      | USART3, Tx D8, Rx D9 and USB Serial Converter A.
      mask init:
      | stm32f4_usart_callback('init');
      mask Help: web(fullfile(waijungdocroot,'stm32f4_usart_setup.htm'), '-browser')
      mask TypeOptions configuration: Setup | Tx | Rx
      mask Callback configuration: stm32f4_usart_callback('configuration');
      mask TypeOptions uartmodule: 1 | 2 | 3 | 4 | 5 | 6
      mask Callback uartmodule: stm32f4_usart_callback('uartmodule');
      mask Callback baudrate: stm32f4_usart_callback('baudrate');
      mask TypeOptions databits: 8
      mask TypeOptions parity: No | Odd | Even
      mask TypeOptions stopbit: 0.5 | 1 | 1.5 | 2
      mask TypeOptions remaptxpin: Not used | A2
      mask TypeOptions remaprxpin: Not used | A3
      mask TypeOptions flowcontrol: None | RTS | CTS | RTS/CTS
      mask Callback flowcontrol: stm32f4_usart_callback('flowcontrol');
      mask TypeOptions remapctspin: Not used | A0
      mask TypeOptions remaprtspin: Not used | A1
      mask Callback advanceoptions: stm32f4_usart_callback('advanceoptions');
      mask TypeOptions rxbuffersize: 16 | 32 | 64 | 128 | 256 | 512 | 1024 | 2048
      mask TypeOptions txbuffersize: 16 | 32 | 64 | 128 | 256 | 512 | 1024 | 2048
      mask TypeOptions transfer: Blocking | Non-Blocking
      mask Callback transfer: stm32f4_usart_callback('transfer');
      mask TypeOptions packetmode: Ascii | Binary | String Buffer
      mask Callback packetmode: stm32f4_usart_callback('packetmode');
      mask Callback binheader: stm32f4_usart_callback('binheader');
      mask Callback binterminator: stm32f4_usart_callback('binterminator');
      mask Callback porttype_double: stm32f4_usart_callback('porttype');
      mask Callback porttype_single: stm32f4_usart_callback('porttype');
      mask Callback porttype_int8: stm32f4_usart_callback('porttype');
      mask Callback porttype_uint8: stm32f4_usart_callback('porttype');
      mask Callback porttype_int16: stm32f4_usart_callback('porttype');
      mask Callback porttype_uint16: stm32f4_usart_callback('porttype');
      mask Callback porttype_int32: stm32f4_usart_callback('porttype');
      mask Callback porttype_uint32: stm32f4_usart_callback('porttype');
      mask Callback asciiformat: stm32f4_usart_callback('asciiformat');
      mask TypeOptions rx_asciiterminator: CR (0x0D - "\r") | LF (0x0A - "\n") | CRLF (0x0D 0x0A - "\r\n")
      mask Callback rx_asciiterminator: stm32f4_usart_callback('rx_asciiterminator');
      mask TypeOptions tx_asciiterminator: CR (0x0D - "\r") | LF (0x0A - "\n") | CRLF (0x0D 0x0A - "\r\n") | None
      mask Callback tx_asciiterminator: stm32f4_usart_callback('tx_asciiterminator');
      mask TypeOptions storagename: <empty>
      mask Callback storagename: stm32f4_usart_callback('storagename');
      mask Callback varname: stm32f4_usart_callback('varname');
      mask Callback sampletime: stm32f4_usart_callback('sampletime');
      mask Callback sampletimestr: stm32f4_usart_callback('sampletimestr');
      mask Callback blockid: stm32f4_usart_callback('blockid');
      mask Display: text(0.5, 0.5, 'Module: USART2_Setup\nBaud (Bps): 5500000\nDMA Buffer: 1024/1024\nTx/Rx Pin: A2/A3','ver','middle','hor','center');
  UART Tx : S-Function  Priority=1  FunctionName=stm32f4_usart  Parameters=configuration,uartmodule,transfer,baudrate,inputtype,outputtype,confstr,binheaderarray,binterminatorarray,asciiheader,asciiterminator,bindatalength,packetmode,varname,sampletime,sampletimestr,blockid  SFunctionDeploymentMode=off  EnableBusSupport=off  mask(stm32f4_usart){configuration=Tx, uartmodule=2, baudrate=115200, databits=8, parity=No, stopbit=1, remaptxpin=Not used, remaprxpin=Not used, flowcontrol=None, remapctspin=Not used, remaprtspin=Not used, advanceoptions=off, rxbuffersize=512, txbuffersize=512, transfer=Blocking, packetmode=Binary, binheader='7E', binterminator='03', porttype_double=0, porttype_single=9, porttype_int8=0, porttype_uint8=0, porttype_int16=0, porttype_uint16=0, porttype_int32=0, porttype_uint32=0, asciiformat='%.2f,%d', rx_asciiterminator=CRLF (0x0D 0x0A - "\r\n"), tx_asciiterminator=CRLF (0x0D 0x0A - "\r\n"), storagename=<empty>, varname=, inputtype=[9  1 1 1 1 1 1 1 1 1], outputtype=[0], binheaderarray=[1 126], binterminatorarray=[1 3], bindatalength=36, asciiheader='%.2f,%d\r\n', asciiterminator=[2 13 10], sampletime=1e-3, sampletimestr=-1, blockid=USARTTransmissionUARTTx, confstr=[ "dummy", "0", "*", "*", "0", "*", "*", "0", "*", "*", "0", "*", "*", "1", "4", "6", "1", "4", "5", "512", "512", "1", "2", "115200", "8", "No", "1", "None", "USART2"], lastmodule=1}
      mask prompts: uartmodule "UART Module"; baudrate "Baud rate (bps)"; databits "Data bits"; stopbit "Stop bit"; remaptxpin "Tx Pin"; remaprxpin "Rx Pin"; flowcontrol "Hardware flow control"; remapctspin "HW Flow control, CTS Pin"; remaprtspin "HW Flow control, RTS Pin"; advanceoptions "Advance options"; rxbuffersize "Rx buffer size (bytes)"; txbuffersize "Tx buffer size (bytes)"; packetmode "Packet mode"; binheader "Binary header (example: '7E 7E')"; binterminator "Binary terminator (example: '03 03')"; porttype_double "Number of data port, type DOUBLE"; porttype_single "Number of data port, type SINGLE"; porttype_int8 "Number of data port, type INT8"; porttype_uint8 "Number of data port, type UINT8"; porttype_int16 "Number of data port, type INT16"; porttype_uint16 "Number of data port, type UINT16"; porttype_int32 "Number of data port, type INT32"; porttype_uint32 "Number of data port, type UINT32"; asciiformat "Ascii format"; rx_asciiterminator "End of packet"; tx_asciiterminator "End of packet"; storagename "Buffer"; varname "Var name"; inputtype "Input data type"; outputtype "Output data type"; binheaderarray "Binary header"; binterminatorarray "Binary terminator"; bindatalength "Binary data length"; asciiheader "Ascii header (printf format)"; asciiterminator "Ascii terminator"; sampletime "Sample time (sec)"; sampletimestr "Compiled sample time (sec) in string"; confstr "Configuration string"; lastmodule "Last module selected"
      mask help:
      | Data type for Ascii format
      | %u, %i, %d, %o, %x: uint32
      | %e, %g, %f: single
      | %c: int8
      mask init:
      | stm32f4_usart_callback('init');
      mask Help: web(fullfile(waijungdocroot,'stm32f4_usart_tx.htm'), '-browser')
      mask TypeOptions configuration: Setup | Tx | Rx
      mask Callback configuration: stm32f4_usart_callback('configuration');
      mask TypeOptions uartmodule: 1 | 2 | 3 | 4 | 5 | 6
      mask Callback uartmodule: stm32f4_usart_callback('uartmodule');
      mask Callback baudrate: stm32f4_usart_callback('baudrate');
      mask TypeOptions databits: 8
      mask TypeOptions parity: No | Odd | Even
      mask TypeOptions stopbit: 0.5 | 1 | 1.5 | 2
      mask TypeOptions remaptxpin: Not used | A9 | B6
      mask TypeOptions remaprxpin: Not used | A10 | B7
      mask TypeOptions flowcontrol: None | RTS | CTS | RTS/CTS
      mask Callback flowcontrol: stm32f4_usart_callback('flowcontrol');
      mask TypeOptions remapctspin: Not used | A11
      mask TypeOptions remaprtspin: Not used | A12
      mask Callback advanceoptions: stm32f4_usart_callback('advanceoptions');
      mask TypeOptions rxbuffersize: 16 | 32 | 64 | 128 | 256 | 512 | 1024 | 2048
      mask TypeOptions txbuffersize: 16 | 32 | 64 | 128 | 256 | 512 | 1024 | 2048
      mask TypeOptions transfer: Blocking | Non-Blocking
      mask Callback transfer: stm32f4_usart_callback('transfer');
      mask TypeOptions packetmode: Ascii | Binary | Binary Vector | String Buffer | Raw Buffer
      mask Callback packetmode: stm32f4_usart_callback('packetmode');
      mask Callback binheader: stm32f4_usart_callback('binheader');
      mask Callback binterminator: stm32f4_usart_callback('binterminator');
      mask Callback porttype_double: stm32f4_usart_callback('porttype');
      mask Callback porttype_single: stm32f4_usart_callback('porttype');
      mask Callback porttype_int8: stm32f4_usart_callback('porttype');
      mask Callback porttype_uint8: stm32f4_usart_callback('porttype');
      mask Callback porttype_int16: stm32f4_usart_callback('porttype');
      mask Callback porttype_uint16: stm32f4_usart_callback('porttype');
      mask Callback porttype_int32: stm32f4_usart_callback('porttype');
      mask Callback porttype_uint32: stm32f4_usart_callback('porttype');
      mask Callback asciiformat: stm32f4_usart_callback('asciiformat');
      mask TypeOptions rx_asciiterminator: CR (0x0D - "\r") | LF (0x0A - "\n") | CRLF (0x0D 0x0A - "\r\n")
      mask Callback rx_asciiterminator: stm32f4_usart_callback('rx_asciiterminator');
      mask TypeOptions tx_asciiterminator: CR (0x0D - "\r") | LF (0x0A - "\n") | CRLF (0x0D 0x0A - "\r\n") | None
      mask Callback tx_asciiterminator: stm32f4_usart_callback('tx_asciiterminator');
      mask TypeOptions storagename: <empty>
      mask Callback storagename: stm32f4_usart_callback('storagename');
      mask Callback varname: stm32f4_usart_callback('varname');
      mask Callback sampletime: stm32f4_usart_callback('sampletime');
      mask Callback sampletimestr: stm32f4_usart_callback('sampletimestr');
      mask Callback blockid: stm32f4_usart_callback('blockid');
      mask Display: text(0.95, 0.5, 'Module: USART2_Tx\nPacket: Binary\nTransfer: Blocking\nTs (sec): -1','ver','middle','hor','right'); port_label('input', 1,'single'); port_label('input', 2,'single'); port_label('input', 3,'single'); port_label('input', 4,'single'); port_label('input', 5,'single'); port_label('input', 6,'single'); port_label('input', 7,'single'); port_label('input', 8,'single'); port_label('input', 9,'single');
  wires:
  X/1 -> UART Tx/1
  U/1 -> Cast1/1
  Theta/1 -> UART Tx/2
  Cast1/1 -> UART Tx/7
  Demux/1 -> UART Tx/3
  Demux/2 -> UART Tx/4
  Demux/3 -> UART Tx/5
  Demux/4 -> UART Tx/6
  Xe/1 -> Cast2/1
  Cast2/1 -> Demux/1
  Ref/1 -> Cast3/1
  Cast3/1 -> Demux1/1
  Demux1/1 -> UART Tx/8
  Demux1/2 -> UART Tx/9

== matlab function Palan_sim/Castint32To2uint16 ==
  data: x output; u input; y output
function [x,y]= castTo2uint16(u)
xy= typecast(u, 'uint16');
x=xy(1);
y=xy(2);
end

== matlab function Palan_sim/Combine To EncoderX ==
  data: x output uint32; u1 input uint8; u2 input uint8; u3 input uint8; u4 input uint8
function x= casttoint32( u1, u2, u3, u4)

x= uint32(u1) + uint32(u2)*256 + uint32(u3)*(256*256) + uint32(u4)*(256*256*256);
end

== matlab function Palan_sim/Combine To EncoderY ==
  data: x output uint32; u1 input uint8; u2 input uint8; u3 input uint8; u4 input uint8
function x= casttoint32( u1, u2, u3, u4)

x= uint32(u1) + uint32(u2)*256 + uint32(u3)*(256*256) + uint32(u4)*(256*256*256);
end

== matlab function Palan_sim/Castint32to2uint16_2 ==
  data: x output; u input; y output
function [x,y]= castTo2uint16(u)
xy= typecast(u, 'uint16');
x=xy(1);
y=xy(2);
end

== matlab function Palan_sim/Combine To EncoderT ==
  data: x output uint16; u1 input uint8; u2 input uint8
function x= casttoint32( u1, u2)

x= uint16(u1) + uint16(u2)*256;
end

== matlab function Palan_sim/Castint16to2uint8_PWM_Y ==
  data: x1 output; u input; x2 output
function [x1,x2]= castTo2uint8(u)
xy= typecast(u, 'uint8');
x1=xy(1);
x2=xy(2);
end

== matlab function Palan_sim/Castint16to2uint8_PWM_X ==
  data: x1 output; u input; x2 output
function [x1,x2]= castTo2uint8(u)
xy= typecast(u, 'uint8');
x1=xy(1);
x2=xy(2);
end

== matlab function Palan_sim/Button2PWM_Y ==
  data: K input; u input; y output
function y = Button2PWM(K,u)
%u i  the button output and is between -100 and  100, you have to mutiply
%it by 120 to obtain a value between -12000 and +12000, i.e., PMW
%admissible values
y = 120*u*int16(K);

== matlab function Palan_sim/Button2PWM_X ==
  data: K input; u input; y output
function y = Button2PWM(K,u)
%u i  the button output and is between -100 and  100, you have to mutiply
%it by 120 to obtain a value between -12000 and +12000, i.e., PMW
%admissible values
y = (120*u)*int16(K);
